simulink subsystem "cart2sphere"  (R2024b)
settings: Solver=VariableStepAuto  StartTime=0.0  StopTime=10.0  RelTol=1e-3
settings Model: Creator=pierb  LastModifiedBy=pierb

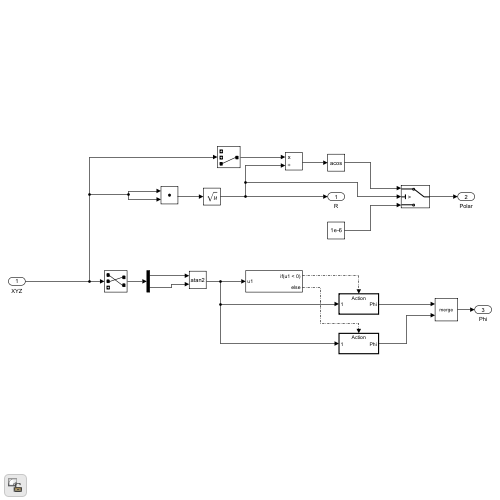
[thumbnail: Simulink's stored preview of the top-level diagram]
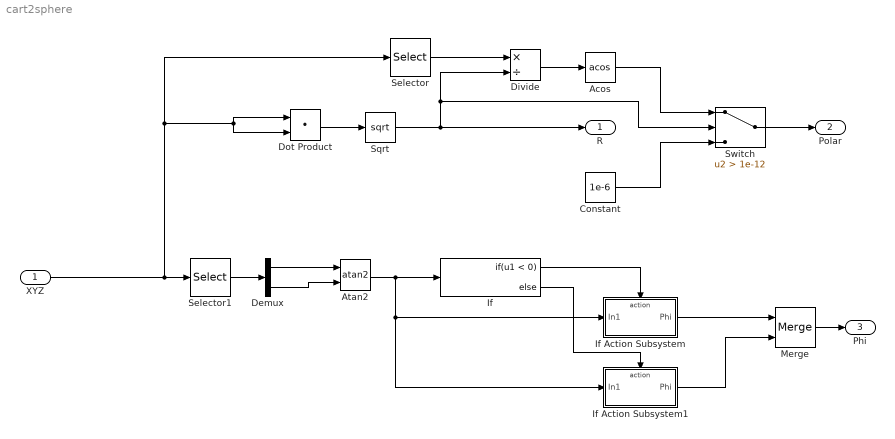
== system cart2sphere ==
  XYZ : Inport
  Acos : Trigonometry  Operator=acos
  Atan2 : Trigonometry  Operator=atan2
  Constant : Constant  Value=1e-6
  Demux : Demux  Outputs=2
  Divide : Product  Inputs=*/
  Dot Product : DotProduct  OutDataTypeStr=Inherit: Inherit via internal rule
  If : If  IfExpression=u1 < 0
  If Action Subsystem : Subsystem  TreatAsAtomicUnit=on
  If Action Subsystem1 : Subsystem  TreatAsAtomicUnit=on
  Merge : Merge
  Selector : Selector  InputPortWidth=3  IndexOptions=Index vector (dialog)  Indices=3  OutputSizes=1
  Selector1 : Selector  InputPortWidth=3  IndexOptions=Index vector (dialog)  Indices=[2 1]  OutputSizes=1
  Sqrt : Sqrt
  Switch : Switch  Criteria=u2 > Threshold  Threshold=1e-12  SaturateOnIntegerOverflow=off  InputSameDT=off
  R : Outport
  Polar : Outport  Port=2
  Phi : Outport  Port=3
  wires:
  Dot Product/1 -> Sqrt/1
  Sqrt/1 -> R/1, Switch/2, Divide/2
  XYZ/1 -> Dot Product/2, Dot Product/1, Selector/1, Selector1/1
  Switch/1 -> Polar/1
  Constant/1 -> Switch/3
  Selector/1 -> Divide/1
  Divide/1 -> Acos/1
  Acos/1 -> Switch/1
  Selector1/1 -> Demux/1
  Demux/1 -> Atan2/1
  Demux/2 -> Atan2/2
  Atan2/1 -> If/1, If Action Subsystem/1(In1), If Action Subsystem1/1(In1)
  If/1 -> If Action Subsystem/Action
  Merge/1 -> Phi/1
  If Action Subsystem/1(Phi) -> Merge/1
  If/2 -> If Action Subsystem1/Action
  If Action Subsystem1/1(Phi) -> Merge/2

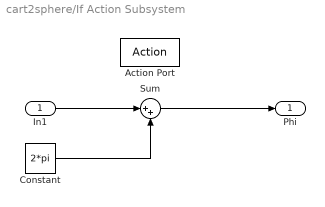
== system cart2sphere/If Action Subsystem ==
  In1 : Inport
  Action Port : ActionPort
  Constant : Constant  Value=2*pi
  Sum : Sum  Inputs=|++
  Phi : Outport
  wires:
  Sum/1 -> Phi/1
  In1/1 -> Sum/1
  Constant/1 -> Sum/2

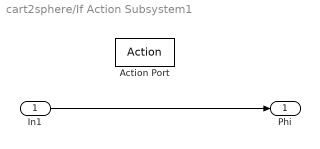
== system cart2sphere/If Action Subsystem1 ==
  In1 : Inport
  Action Port : ActionPort
  Phi : Outport
  wires:
  In1/1 -> Phi/1
